simulink model "TP10_Examen_essuie_glaces_automatiques_stateflow"  (R2022b)
settings: Solver=VariableStepAuto  StartTime=0.0  StopTime=inf  RelTol=1e-3
settings Model: Creator=HP  LastModifiedBy=HP

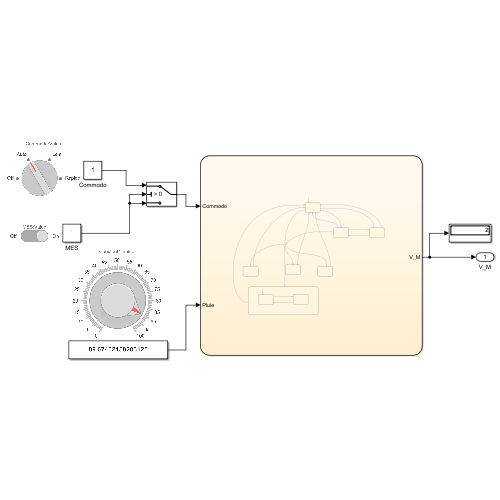
[thumbnail: Simulink's stored preview of the top-level diagram]
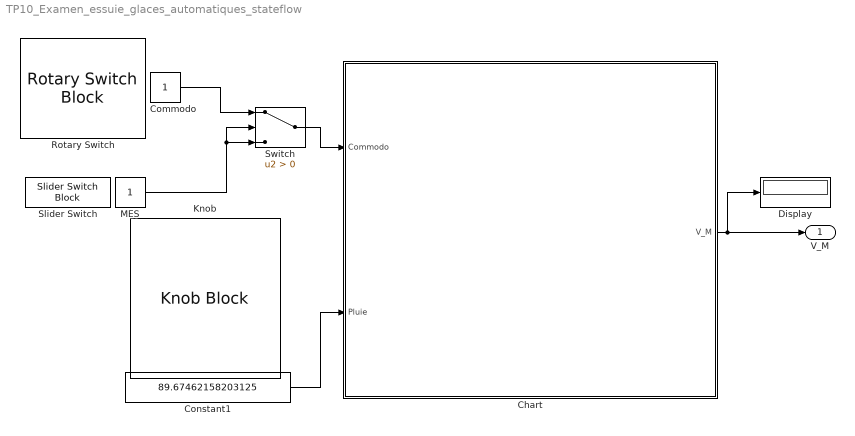
== system TP10_Examen_essuie_glaces_automatiques_stateflow ==
  Chart : Stateflow chart  TreatAsAtomicUnit=on
  Commodo : Constant
  Constant1 : Constant  Value=89.67462158203125
  Display : Display
  Knob : KnobBlock
  MES : Constant
  Rotary Switch : RotarySwitchBlock
      settings: Values={{'Off', 'Auto', 'Lent', 'Rapide'}, [0 1 2 3]}
  Slider Switch : SliderSwitchBlock
      settings: Values={{'Off', 'On'}, [0 1]}
  Switch : Switch  Criteria=u2 > Threshold  SaturateOnIntegerOverflow=off  InputSameDT=off
  V_M : Outport
  wires:
  Constant1/1 -> Chart/2(Pluie)
  Switch/1 -> Chart/1(Commodo)
  MES/1 -> Switch/2, Switch/3
  Chart/1(V_M) -> Display/1, V_M/1
  Commodo/1 -> Switch/1

== stateflow chart TP10_Examen_essuie_glaces_automatiques_stateflow/Chart ==
  state repos
    entry:
    V_M = 0;
  state manuel_Lent
    entry:
    V_M = 1;
  state manuel_rapide
    entry:
    V_M = 2;
  state auto_lent
    entry:
    V_M = 1;
  state auto_repos
    entry:
    V_M = 0;
  state auto_rapide
    entry:
    V_M = 2;
  state faible_pluie
    state repos5
      entry:
      V_M = 1;
    state repos6
      entry:
      V_M = 0;
    (default) -> repos5
    repos5 -> repos6 : [after(1, sec)]
    repos6 -> repos5 : [after(3, sec)]
  (default) -> repos
  manuel_rapide -> repos [order 2] : [Commodo ~= 3]
  faible_pluie -> repos : [Commodo ~= 1 || Pluie < 10 || Pluie >= 50]
  auto_repos -> repos : [Commodo ~= 1 || Pluie > 10]
  repos -> manuel_rapide [order 3] : [Commodo == 3]
  repos -> (junction 11) [order 1] : [Commodo == 1]
  repos -> manuel_Lent [order 2] : [Commodo == 2]
  auto_lent -> repos : [Pluie < 50 || Pluie >= 80 || Commodo ~= 1]
  manuel_Lent -> repos [order 3] : [Commodo ~= 2]
  auto_rapide -> repos : [Pluie < 80 || Commodo ~= 1]
  manuel_Lent -> manuel_rapide [order 1] : [Commodo == 3]
  manuel_Lent -> (junction 11) [order 2] : [Commodo == 1]
  manuel_rapide -> manuel_Lent [order 1] : [Commodo == 2]
  (junction 11) -> auto_repos [order 1] : [Pluie <= 10]
  (junction 11) -> auto_rapide [order 3] : [Pluie >= 80]
  (junction 11) -> auto_lent [order 2] : [Pluie >= 50 && Pluie < 80 ]
  (junction 11) -> faible_pluie [order 4] : [Pluie >= 10 && Pluie < 50]
  data: Commodo input; Pluie input; V_M output
